simulink model "ARDroneReplay_5"  (R2025b)
settings: Solver=ode1  StartTime=0.0  StopTime=45.145  FixedStep=sampleTime  RelTol=1e-3  EnableMultiTasking=on
values from neighbouring files (symbols this model uses):
  P0 = blkdiag(1e-3*eye(3), 0.05^2*eye(3))    [setup_5.m]
  Q = diag([Q_phi, Q_theta])    [setup_4_1.m]    (also in setup_4_4.m; setup_5.m = kq*Q_acc)
  R = diag([R_p, R_q])    [setup_4_1.m]    (also in setup_4_4.m = diag([R_p, R_q, R_bp, R_bq]); setup_5.m = blkdiag(R_gyro, kb*R_gyro))
  sampleTime = 1/200    (= 0.005)    [setup_4_1.m]    (also in setup_4_4.m; setup_5.m)
  x0 = [0; 0; 1; 0; 0; 0]    [setup_5.m]
libraries: ARBlocks x2
settings Model: ExtModeTrigDuration=100000  Creator=Paul  LastModifiedBy=caio
settings SolverCC: AlgebraicLoopSolver=TrustRegion
settings DataIOCC: LimitDataPoints=on  SaveFormat=Array  SignalLoggingSaveFormat=ModelDataLogs  ReturnWorkspaceOutputs=off  TimeSaveName=time
settings OptimizationCC: ExpressionDepthLimit=2147483647.0  InitFltsAndDblsToZero=on
settings DebuggingCC: UnderspecifiedInitializationDetection=Classic  MergeDetectMultiDrivingBlocksExec=none  SolverPrmCheckMsg=warning  FcnCallInpInsideContextMsg=warning  UnconnectedInputMsg=warning  UnconnectedOutputMsg=warning  UnconnectedLineMsg=warning  StateNameClashWarn=warning  SFUnexpectedBacktrackingDiag=warning  SFNoUnconditionalDefaultTransitionDiag=warning  SFExecutionAtInitializationDiag=none  ArithmeticOperatorsInVariantConditions=warning
settings HardwareCC: ProdBitPerLong=64.0  ProdHWDeviceType=Intel->x86-64 (Linux 64)
settings ModelReferenceCC: EnableRefExpFcnMdlSchedulingChecks=on  PropagateSignalLabelsOutOfModel=off
settings SFSimCC: SimUseLocalCustomCode=off  CustomCodeUndefinedFunction=UseInterfaceOnly
settings RTWCC: SystemTargetFile=sldrt.tlc  TemplateMakefile=sldrt.tmf  RTWUseLocalCustomCode=off  RTWCompilerOptimization=on  GPUComputeCapability=3.5  Description=Simulink Desktop Real-Time
settings CodeAppCC: MaxIdLength=95.0  StateflowObjectComments=on
settings SimulinkDesktopRealTimeCC: ExtModeTransport=0.0  ExtModeStaticAllocSize=1000000.0  TargetLibSuffix=_sldrt.a  TargetPreCompLibLocation=/home/caio/.local/share/MATLAB/R2025b/toolbox/sldrt/lib/glnxa64  TargetLangStandard=C89/C90 (ANSI)  MultiwordLength=2048.0  DynamicStringBufferSize=256.0  ParMdlRefBuildCompliant=on  PreserveMATLABNamespacesInGeneratedCode=on  SubcomponentCodeInterfacePackaging=Reusable function  SupportVariableSizeSignals=off
settings ConfigComp: CovMetricSettings=dw  CovSaveCumulativeToWorkspaceVar=on  CovSaveSingleToWorkspaceVar=on  CovExternalEMLEnable=off

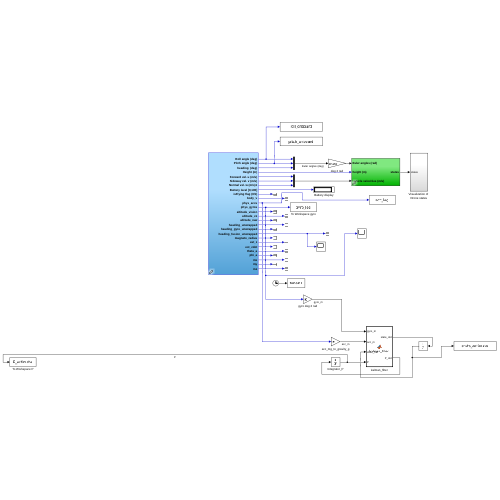
[thumbnail: Simulink's stored preview of the top-level diagram]
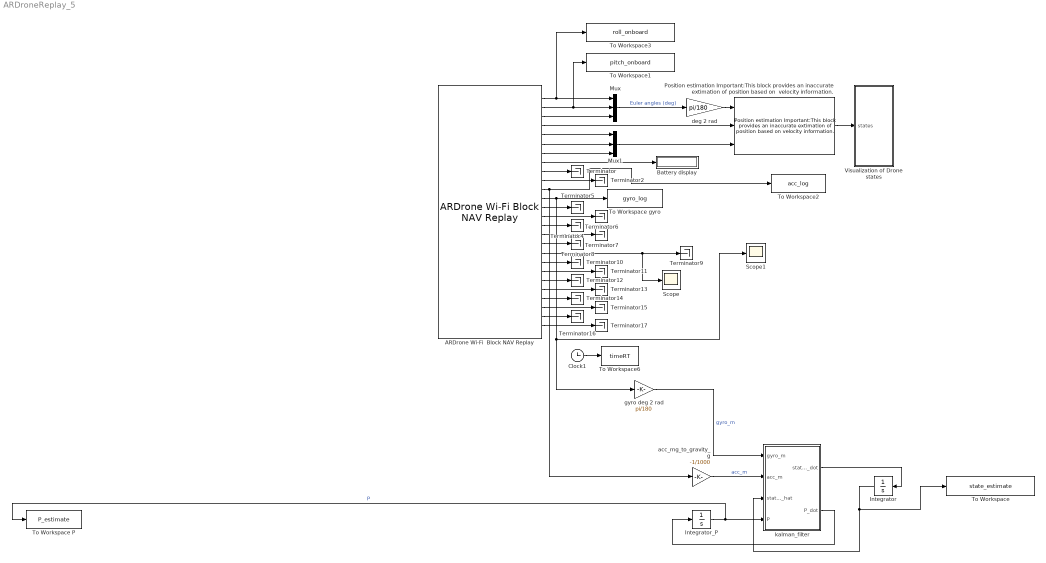
== system ARDroneReplay_5 ==
  ARDrone Wi-Fi  Block NAV Replay : ARBlocks/ARDrone Wi-Fi  Block NAV Replay  SystemSampleTime=-1  VariantActivationTime=update diagram  EmptyChoice=off  PassThrough=off  PassThroughVariantControl=(default)  EmptyChoiceVariantControl=(default)  AllowFlexibleInterface=on  Latency=0  AutoFrameSizeCalculation=off
  Battery display : Display
  Clock1 : Clock
  Integrator : Integrator  InitialCondition=x0
  Integrator_P : Integrator  InitialCondition=P0
  Mux : Mux  Inputs=3
  Mux1 : Mux  Inputs=3
  "Position estimation Important:This block provides an inaccurate extimation of position based on  velocity information. " : ARBlocks/Position estimation Important:This block provides an  inaccurate extimation of position  based on  velocity information.   SystemSampleTime=-1  VariantActivationTime=update diagram  EmptyChoice=off  PassThrough=off  PassThroughVariantControl=(default)  EmptyChoiceVariantControl=(default)  AllowFlexibleInterface=on  Latency=0  AutoFrameSizeCalculation=off
  Scope : Scope
      settings: ActiveDisplayYMinimum=-0.58202  ActiveDisplayYMaximum=1.32261
  Scope1 : Scope
      settings: ActiveDisplayYMinimum=-0.28836918249726295  ActiveDisplayYMaximum=0.25480991974473
  Terminator{,2,4..17} (16 alike) : Terminator
  To Workspace : ToWorkspace  VariableName=state_estimate  SaveFormat=Structure With Time  SampleTime=-1
  To Workspace P : ToWorkspace  VariableName=P_estimate  SaveFormat=Structure With Time  SampleTime=-1
  To Workspace gyro : ToWorkspace  VariableName=gyro_log  SaveFormat=Structure With Time  SampleTime=-1
  To Workspace1 : ToWorkspace  VariableName=pitch_onboard  SaveFormat=Structure With Time  SampleTime=-1
  To Workspace2 : ToWorkspace  VariableName=acc_log  SaveFormat=Structure With Time  SampleTime=-1
  To Workspace3 : ToWorkspace  VariableName=roll_onboard  SaveFormat=Structure With Time  SampleTime=-1
  To Workspace6 : ToWorkspace  VariableName=timeRT  SampleTime=sampleTime
  Visualization of Drone states : Subsystem
  acc_mg_to_gravity_g : Gain  Gain=-1/1000
  deg 2 rad : Gain  Gain=pi/180
  gyro deg 2 rad : Gain  Gain=pi/180
  kalman_filter : MATLAB Function  TreatAsAtomicUnit=on
  wires:
  ARDrone Wi-Fi  Block NAV Replay/1 -> To Workspace3/1, Mux/1
  ARDrone Wi-Fi  Block NAV Replay/2 -> To Workspace1/1, Mux/2
  ARDrone Wi-Fi  Block NAV Replay/5 -> Mux1/1
  ARDrone Wi-Fi  Block NAV Replay/6 -> Mux1/2
  ARDrone Wi-Fi  Block NAV Replay/7 -> Mux1/3
  Mux/1 -> deg 2 rad/1  "Euler angles (deg)"
  ARDrone Wi-Fi  Block NAV Replay/8 -> Battery display/1
  "Position estimation Important:This block provides an inaccurate extimation of position based on  velocity information. "/1 -> Visualization of Drone states/1(states)
  deg 2 rad/1 -> "Position estimation Important:This block provides an inaccurate extimation of position based on  velocity information. "/1
  ARDrone Wi-Fi  Block NAV Replay/4 -> "Position estimation Important:This block provides an inaccurate extimation of position based on  velocity information. "/2
  Mux1/1 -> "Position estimation Important:This block provides an inaccurate extimation of position based on  velocity information. "/3
  ARDrone Wi-Fi  Block NAV Replay/3 -> Mux/3
  ARDrone Wi-Fi  Block NAV Replay/9 -> Terminator/1
  Clock1/1 -> To Workspace6/1
  ARDrone Wi-Fi  Block NAV Replay/15 -> Terminator4/1
  ARDrone Wi-Fi  Block NAV Replay/10 -> Terminator2/1
  ARDrone Wi-Fi  Block NAV Replay/13 -> Terminator5/1
  ARDrone Wi-Fi  Block NAV Replay/14 -> Terminator6/1
  ARDrone Wi-Fi  Block NAV Replay/17 -> Terminator8/1
  ARDrone Wi-Fi  Block NAV Replay/16 -> Terminator7/1
  ARDrone Wi-Fi  Block NAV Replay/19 -> Terminator10/1
  ARDrone Wi-Fi  Block NAV Replay/18 -> Scope/1, Terminator9/1
  ARDrone Wi-Fi  Block NAV Replay/21 -> Terminator12/1
  ARDrone Wi-Fi  Block NAV Replay/20 -> Terminator11/1
  ARDrone Wi-Fi  Block NAV Replay/23 -> Terminator14/1
  ARDrone Wi-Fi  Block NAV Replay/22 -> Terminator13/1
  ARDrone Wi-Fi  Block NAV Replay/25 -> Terminator16/1
  ARDrone Wi-Fi  Block NAV Replay/24 -> Terminator15/1
  ARDrone Wi-Fi  Block NAV Replay/26 -> Terminator17/1
  kalman_filter/1(state_dot) -> Integrator/1
  ARDrone Wi-Fi  Block NAV Replay/12 -> gyro deg 2 rad/1, Scope1/1, To Workspace gyro/1
  Integrator/1 -> To Workspace/1, kalman_filter/3(state_hat)
  gyro deg 2 rad/1 -> kalman_filter/1(gyro_m)  "gyro_m"
  kalman_filter/2(P_dot) -> Integrator_P/1
  Integrator_P/1 -> To Workspace P/1, kalman_filter/4(P)  "P"
  acc_mg_to_gravity_g/1 -> kalman_filter/2(acc_m)  "acc_m"
  ARDrone Wi-Fi  Block NAV Replay/11 -> To Workspace2/1, acc_mg_to_gravity_g/1

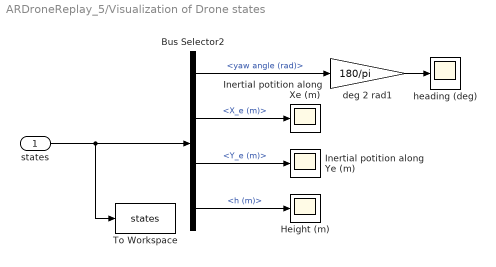
== system ARDroneReplay_5/Visualization of Drone states ==
  states : Inport
  Bus Selector2 : BusSelector  OutputSignals=yaw angle (rad),X_e (m),Y_e (m),h (m)
  Height (m) : Scope
      settings: ActiveDisplayYMinimum=-0.15212  ActiveDisplayYMaximum=1.36913  DataLoggingMaxPoints=500000  DataLoggingVariableName=ScopeData5
  Inertial potition along Xe (m) : Scope
      settings: ActiveDisplayYMinimum=-0.49449  ActiveDisplayYMaximum=0.46559  DataLoggingMaxPoints=500000  DataLoggingVariableName=ScopeData3
  Inertial potition along Ye (m) : Scope
      settings: ActiveDisplayYMinimum=-0.28577  ActiveDisplayYMaximum=0.69906  DataLoggingMaxPoints=500000  DataLoggingVariableName=ScopeData4
  To Workspace : ToWorkspace  VariableName=states  SaveFormat=Structure With Time  SampleTime=-1
  deg 2 rad1 : Gain  Gain=180/pi
  heading (deg) : Scope
      settings: ActiveDisplayYMinimum=-139.82962  ActiveDisplayYMaximum=15.53662  DataLoggingMaxPoints=500000  DataLoggingVariableName=ScopeData2
  wires:
  states/1 -> To Workspace/1, Bus Selector2/1
  Bus Selector2/1 -> deg 2 rad1/1  "<yaw angle (rad)>"
  Bus Selector2/2 -> Inertial potition along Xe (m)/1  "<X_e (m)>"
  Bus Selector2/3 -> Inertial potition along Ye (m)/1  "<Y_e (m)>"
  Bus Selector2/4 -> Height (m)/1  "<h (m)>"
  deg 2 rad1/1 -> heading (deg)/1

== matlab function ARDroneReplay_5/kalman_filter ==
  data: gyro_m input; state_dot output; acc_m input; state_hat input; P input; Q parameter; P_dot output; R parameter
function [state_dot, P_dot] = kalman_filter(gyro_m, acc_m, state_hat, P, Q, R)
    % Kalman filter for the nominal system (2) of Batista et al., as an LTV system
    %   state_hat = [x; b]   x: gravity direction in {B} (g), b: gyro bias (rad/s)
    %   gyro_m: rate gyro (rad/s)      acc_m: gravity measured in {B} (g)
    %   R: process noise (gyro, bias)  Q: measurement noise (accelerometer)
    A = [-skew(gyro_m), -skew(acc_m); zeros(3, 6)];
    G = [-skew(acc_m), zeros(3); zeros(3), eye(3)];
    C = [eye(3), zeros(3)];
    K = P*C'/Q;
    state_dot = A*state_hat + K*(acc_m - C*state_hat);
    P_dot     = A*P + P*A' + G*R*G' - K*Q*K';
end

function S = skew(v)
    S = [0 -v(3) v(2); v(3) 0 -v(1); -v(2) v(1) 0];
end
